simulink subsystem "Subsys_Conv_Electrical_Part_imperix_SPS"  (R2022b)
settings: Solver=VariableStepAuto  StartTime=0.0  StopTime=10.0  RelTol=1e-3
model mask{S_n=27e3, f_n=50, V_n_phph=400, V_n_grid_phph=400, V_n_dc=800, L_filter_conv_pu=[ 0.005 0.06257 ], C_filter_pu=[ 0.08437 0.03724 ], R_snubber_pu=5e6, R_on_pu=8.437e-3, C_dc_pu=5.826, P_dc_max=30e3, K_p_DC=20, K_i_DC=50}
  mask prompts: S_n "Nominal Apparent Power [VA]"; f_n "Nominal Frequency [Hz]"; V_n_phph "Nominal Converter Voltage (rms, ph-ph) [V]"; V_n_grid_phph "Nominal Grid Voltage (rms, ph-ph) [V]"; V_n_dc "DC-link voltage [V]"; L_filter_conv_pu "Impedance of Converter-Side-Inductor [ R L ] (p.u.)"; C_filter_pu "Impedance of Filter Capacitor [ R C ] (p.u.)"; R_snubber_pu "Snubber Resistance for Ideal Switches (pu)"; R_on_pu "On-State Resistance of Ideal Switches (pu)"; C_dc_pu "Capacitance of DC-link capacitors (total) (pu)"; P_dc_max "Maximum power of DC voltage source [W]"; K_p_DC "Current controller proportional gain (pu)"; K_i_DC "Current controller integral gain (pu/s)"
libraries: spsThreePhaseVIMeasurementLib x4, spsThreePhaseSeriesRLCBranchLib x3, spsSeriesRLCBranchLib x2, spsVoltageMeasurementLib x2, spsGroundLib x2, spsBreakerLib x2, spsThreePhaseBreakerLib x2, spsCurrentMeasurementLib x1, spsControlledCurrentSourceLib x1, slpidlib x1, spsUniversalBridgeLib x1
settings Model: Creator=winkens  LastModifiedBy=winkens
settings SolverCC: AlgebraicLoopSolver=TrustRegion
settings DebuggingCC: UnconnectedInputMsg=warning  UnconnectedOutputMsg=warning  UnconnectedLineMsg=warning  SFMachineParentedDataDiag=warning
settings ModelReferenceCC: EnableRefExpFcnMdlSchedulingChecks=on
settings RTWCC: DLArmComputeVersion=19.05

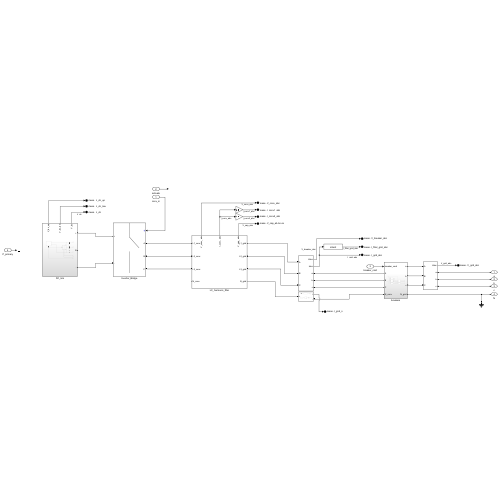
[thumbnail: Simulink's stored preview of the top-level diagram]
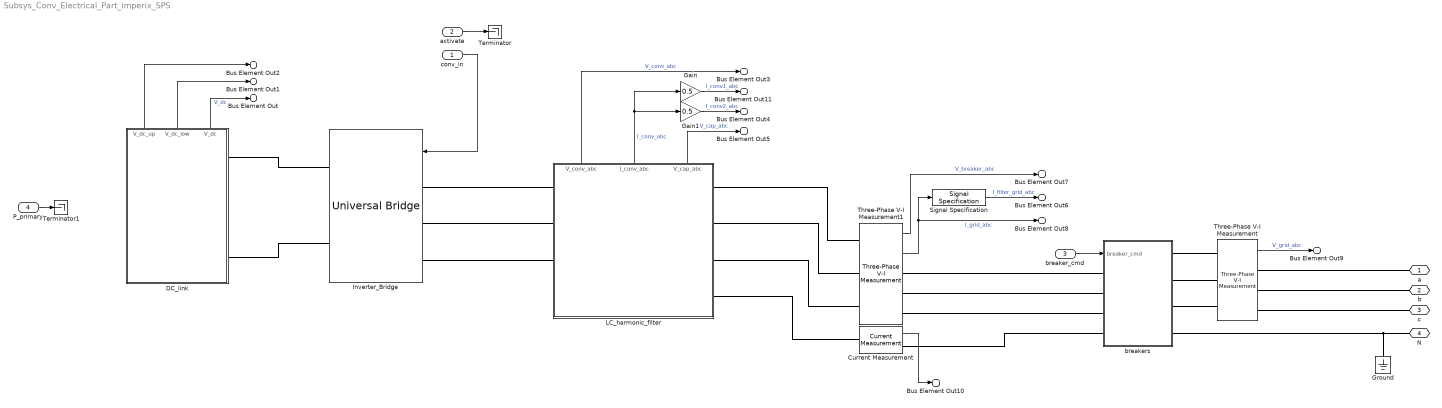
== system Subsys_Conv_Electrical_Part_imperix_SPS ==
  conv_in : Inport
  activate : Inport  Port=2
  breaker_cmd : Inport  Port=3
  P_primary : Inport  Port=4
  Current Measurement : spsCurrentMeasurementLib/Current Measurement  PhasorSimulation=off  OutputType=Complex  PSBequivalent=0
  DC_link : Subsystem  VariantControl=(default)
      settings: PortSchema="{\"entries\":[{\"content\":{\"sides\":[{\"content\":{\"connectorIds\":[]},\"type\":\"ConnectorPlacement.EquallySpacedRectSide\",\"uuid\":\"14f4955d-76e2-48f7-8123-585826302dd3\"},{\"content\":{\"connectorIds\":[\"RConn1\",\"RConn2\",\"RConn3\"],\"side\":\"RIGHT\"},\"type\":\"ConnectorPlacement.EquallySpacedRectSide\",\"uuid\":\"28c9ddee-fc07-46e8-b9fa-376576ca9eeb\"},{\"content\":{\"connectorIds\":[\"Out1\",\"Out2\",\"Out3\"],\"side\":\"TOP\"},\"type\":\"ConnectorPlacement.EquallySpacedRectSide\",\"uuid\":\"aa37790b-34b3-4fc7-a446-818c7dbc2b0a\"},{\"content\":{\"connectorIds\":[],\"side\":\"HIDDEN\"},\"type\":\"ConnectorPlacement.EquallySpacedRectSide\",\"uuid\":\"98235a86-067a-4efe-b161-de7bc0b16115\"}]},\"type\":\"ConnectorPlacement.EquallySpacedConnector\",\"uuid\":\"03b86b37-ee57-4f73-9f3c-01f441a0fa47\"}],\"packageUris\":[\"http://schema.mathworks.com/mf0/Connector/R2020b\"],\"version\":\"1.0\"}"
  Gain : Gain  Gain=0.5
  Gain1 : Gain  Gain=0.5
  Ground : spsGroundLib/Ground  LConnTagsString=a
  Inverter_Bridge : spsUniversalBridgeLib/Universal Bridge  Arms=3  SnubberResistance=R_snubber_pu*V_n_phph*V_n_phph/S_n  SnubberCapacitance=inf  Device=Ideal Switches  Ron=R_on_pu*V_n_phph*V_n_phph/S_n  Lon=0  ForwardVoltages="[  0  0  ]"  ForwardVoltage=0  GTOparameters=[ 10e-6 , 20e-6 ]  IGBTparameters=[ 1e-6 , 2e-6 ]  Measurements=None  Measurements_2=None  converterType=Rectifier
  LC_harmonic_filter : Subsystem
      settings: PortSchema="{\"entries\":[{\"content\":{\"sides\":[{\"content\":{\"connectorIds\":[\"LConn1\",\"LConn2\",\"LConn3\",\"LConn4\"]},\"type\":\"ConnectorPlacement.EquallySpacedRectSide\",\"uuid\":\"80edb88e-7f34-4d55-b68e-78bf26c6ccee\"},{\"content\":{\"connectorIds\":[\"RConn1\",\"RConn2\",\"RConn3\",\"RConn4\"],\"side\":\"RIGHT\"},\"type\":\"ConnectorPlacement.EquallySpacedRectSide\",\"uuid\":\"4bc9f7f6-7a52-4676-a444-e90f3617f1ed\"},{\"content\":{\"connectorIds\":[\"Out1\",\"Out2\",\"Out3\"],\"side\":\"TOP\"},\"type\":\"ConnectorPlacement.EquallySpacedRectSide\",\"uuid\":\"b4b56f07-3fcd-4b33-a68a-5af0641c9948\"},{\"content\":{\"connectorIds\":[],\"side\":\"HIDDEN\"},\"type\":\"ConnectorPlacement.EquallySpacedRectSide\",\"uuid\":\"916e6694-bfd6-4ec0-aa17-f6867d02ef86\"}]},\"type\":\"ConnectorPlacement.EquallySpacedConnector\",\"uuid\":\"94bee9f6-0fe3-4fcb-8152-95dcfa33148b\"}],\"packageUris\":[\"http://schema.mathworks.com/mf0/Connector/R2020b\"],\"version\":\"1.0\"}"
  Signal Specification : SignalSpecification
  Terminator : Terminator
  Terminator1 : Terminator
  Three-Phase V-I Measurement : spsThreePhaseVIMeasurementLib/Three-Phase V-I Measurement  VoltageMeasurement=phase-to-ground  SetLabelV=off  LabelV=Vabc  Vpu=off  VpuLL=off  CurrentMeasurement=no  SetLabelI=off  LabelI=Iabc  Ipu=off  Pbase=100e6  Vbase=500e3  OutputType=Complex  PhasorSimulation=off  PSBequivalent=0
  Three-Phase V-I Measurement1 : spsThreePhaseVIMeasurementLib/Three-Phase V-I Measurement  VoltageMeasurement=phase-to-ground  SetLabelV=off  LabelV=Vabc  Vpu=off  VpuLL=off  CurrentMeasurement=yes  SetLabelI=off  LabelI=Iabc  Ipu=off  Pbase=100e6  Vbase=500e3  OutputType=Complex  PhasorSimulation=off  PSBequivalent=0
  breakers : Subsystem
  a : PMIOPort  Side=Right
  b : PMIOPort  Port=2  Side=Right
  c : PMIOPort  Port=3  Side=Right
  N : PMIOPort  Port=4  Side=Right
  Bus Element Out : Outport  PortName=meas  Element=V_dc
  Bus Element Out1 : Outport  PortName=meas  Element=V_dc_low
  Bus Element Out2 : Outport  PortName=meas  Element=V_dc_up
  Bus Element Out3 : Outport  PortName=meas  Element=V_conv_abc
  Bus Element Out4 : Outport  PortName=meas  Element=I_conv2_abc
  Bus Element Out5 : Outport  PortName=meas  Element=V_cap_ab-bc-ca
  Bus Element Out6 : Outport  PortName=meas  Element=I_filter_grid_abc
  Bus Element Out7 : Outport  PortName=meas  Element=V_breaker_abc
  Bus Element Out8 : Outport  PortName=meas  Element=I_grid_abc
  Bus Element Out10 : Outport  PortName=meas  Element=I_grid_n
  Bus Element Out9 : Outport  PortName=meas  Element=V_grid_abc
  Bus Element Out11 : Outport  PortName=meas  Element=I_conv1_abc
  wires:
  Three-Phase V-I Measurement1/2 -> Signal Specification/1, Bus Element Out8/1  "I_grid_abc"
  Three-Phase V-I Measurement1/1 -> Bus Element Out7/1  "V_breaker_abc"
  LC_harmonic_filter/2(I_conv_abc) -> Gain/1, Gain1/1  "I_conv_abc"
  LC_harmonic_filter/3(V_cap_abc) -> Bus Element Out5/1  "V_cap_abc"
  DC_link/3(V_dc) -> Bus Element Out/1  "V_dc"
  Three-Phase V-I Measurement/1 -> Bus Element Out9/1  "V_grid_abc"
  LC_harmonic_filter/1(V_conv_abc) -> Bus Element Out3/1  "V_conv_abc"
  P_primary/1 -> Terminator1/1
  activate/1 -> Terminator/1
  conv_in/1 -> Inverter_Bridge/1
  Signal Specification/1 -> Bus Element Out6/1  "I_filter_grid_abc"
  DC_link/2(V_dc_low) -> Bus Element Out1/1
  DC_link/1(V_dc_up) -> Bus Element Out2/1
  breaker_cmd/1 -> breakers/1(breaker_cmd)
  Current Measurement/1 -> Bus Element Out10/1
  Gain1/1 -> Bus Element Out4/1  "I_conv2_abc"
  Gain/1 -> Bus Element Out11/1  "I_conv1_abc"
  connections:
  Ground/LConn1 -- breakers/RConn4 -- N/RConn1
  DC_link/RConn1 -- Inverter_Bridge/RConn1
  DC_link/RConn3 -- Inverter_Bridge/RConn2
  Three-Phase V-I Measurement/RConn2 -- b/RConn1
  Three-Phase V-I Measurement/RConn1 -- a/RConn1
  LC_harmonic_filter/LConn3 -- Inverter_Bridge/LConn3
  Three-Phase V-I Measurement/RConn3 -- c/RConn1
  LC_harmonic_filter/LConn1 -- Inverter_Bridge/LConn1
  LC_harmonic_filter/LConn2 -- Inverter_Bridge/LConn2
  Three-Phase V-I Measurement1/LConn1 -- LC_harmonic_filter/RConn1
  Three-Phase V-I Measurement1/LConn2 -- LC_harmonic_filter/RConn2
  Three-Phase V-I Measurement1/LConn3 -- LC_harmonic_filter/RConn3
  Three-Phase V-I Measurement/LConn1 -- breakers/RConn1
  Three-Phase V-I Measurement1/RConn1 -- breakers/LConn1
  Three-Phase V-I Measurement/LConn2 -- breakers/RConn2
  Three-Phase V-I Measurement1/RConn2 -- breakers/LConn2
  Current Measurement/LConn1 -- LC_harmonic_filter/RConn4
  Three-Phase V-I Measurement/LConn3 -- breakers/RConn3
  Three-Phase V-I Measurement1/RConn3 -- breakers/LConn3
  Current Measurement/RConn1 -- breakers/LConn4

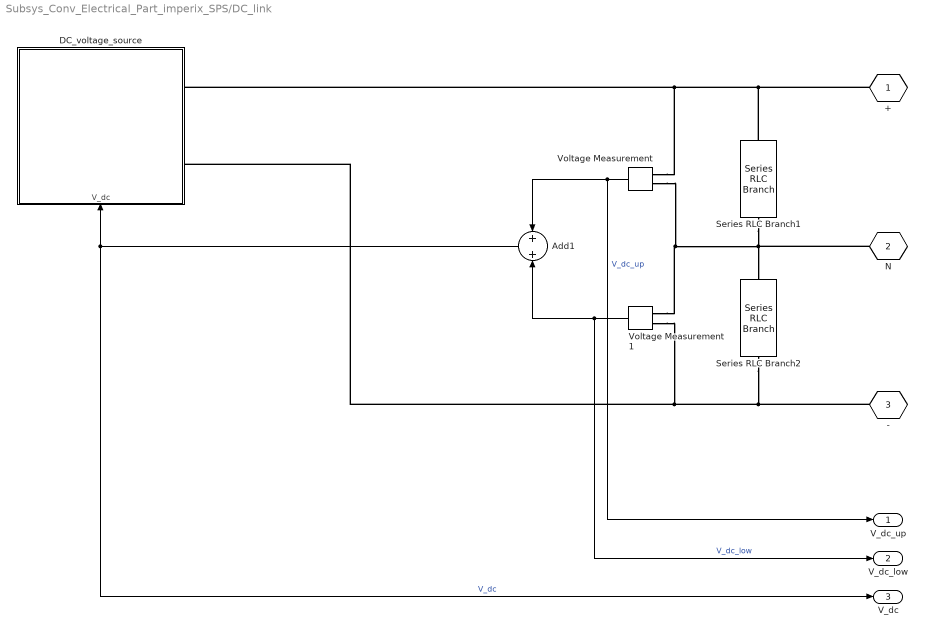
== system Subsys_Conv_Electrical_Part_imperix_SPS/DC_link ==
  Add1 : Sum  Inputs=+|+
  DC_voltage_source : Subsystem
      settings: PortSchema="{\"entries\":[{\"content\":{\"sides\":[{\"content\":{\"connectorIds\":[]},\"type\":\"ConnectorPlacement.EquallySpacedRectSide\",\"uuid\":\"a61cbdc0-cd1f-4d97-8c38-69a1c66b7135\"},{\"content\":{\"connectorIds\":[\"RConn1\",\"RConn2\"],\"side\":\"RIGHT\"},\"type\":\"ConnectorPlacement.EquallySpacedRectSide\",\"uuid\":\"763bad63-06eb-40cb-9b7c-68a57cfbd908\"},{\"content\":{\"connectorIds\":[],\"side\":\"TOP\"},\"type\":\"ConnectorPlacement.EquallySpacedRectSide\",\"uuid\":\"0a61cfd4-8f0a-43bb-bfe4-f1bce7526c22\"},{\"content\":{\"connectorIds\":[\"In1\"],\"side\":\"BOTTOM\"},\"type\":\"ConnectorPlacement.EquallySpacedRectSide\",\"uuid\":\"8fa3c57f-1077-4c84-877b-6ab8e99a2e0f\"},{\"content\":{\"connectorIds\":[],\"side\":\"HIDDEN\"},\"type\":\"ConnectorPlacement.EquallySpacedRectSide\",\"uuid\":\"ed7d5b32-63bb-486f-8710-8f53ee798462\"}]},\"type\":\"ConnectorPlacement.EquallySpacedConnector\",\"uuid\":\"0213af1d-3c14-41a0-aa43-0a8d2de349d1\"}],\"packageUris\":[\"http://schema.mathworks.com/mf0/Connector/R2020b\"],\"version\":\"1.0\"}"
  Series RLC Branch1 : spsSeriesRLCBranchLib/Series RLC Branch  LConnTagsString=__new0  RConnTagsString=__new0  BranchType=C  Resistance=1  Inductance=1e-3  SetiL0=off  InitialCurrent=0  Capacitance=2*C_dc_pu*S_n/(2*pi*f_n*V_n_phph*V_n_phph)  Setx0=on  InitialVoltage=V_n_dc/2  Measurements=None
  Series RLC Branch2 : spsSeriesRLCBranchLib/Series RLC Branch  LConnTagsString=__new0  RConnTagsString=__new0  BranchType=C  Resistance=1  Inductance=1e-3  SetiL0=off  InitialCurrent=0  Capacitance=2*C_dc_pu*S_n/(2*pi*f_n*V_n_phph*V_n_phph)  Setx0=on  InitialVoltage=V_n_dc/2  Measurements=None
  Voltage Measurement : spsVoltageMeasurementLib/Voltage Measurement  PhasorSimulation=off  OutputType=Complex  PSBequivalent=0
  Voltage Measurement1 : spsVoltageMeasurementLib/Voltage Measurement  PhasorSimulation=off  OutputType=Complex  PSBequivalent=0
  + : PMIOPort  Tag=PMCPort  Side=Right
  N : PMIOPort  Tag=PMCPort  Port=2  Side=Right
  - : PMIOPort  Tag=PMCPort  Port=3  Side=Right
  V_dc_up : Outport
  V_dc_low : Outport  Port=2
  V_dc : Outport  Port=3
  wires:
  Voltage Measurement/1 -> V_dc_up/1, Add1/1  "V_dc_up"
  Voltage Measurement1/1 -> V_dc_low/1, Add1/2  "V_dc_low"
  Add1/1 -> V_dc/1, DC_voltage_source/1(V_dc)  "V_dc"
  connections:
  Series RLC Branch2/RConn1 -- -/RConn1 -- DC_voltage_source/RConn2 -- Voltage Measurement1/LConn2
  Series RLC Branch1/RConn1 -- Voltage Measurement/LConn2 -- Voltage Measurement1/LConn1 -- Series RLC Branch2/LConn1 -- N/RConn1
  +/RConn1 -- Series RLC Branch1/LConn1 -- DC_voltage_source/RConn1 -- Voltage Measurement/LConn1

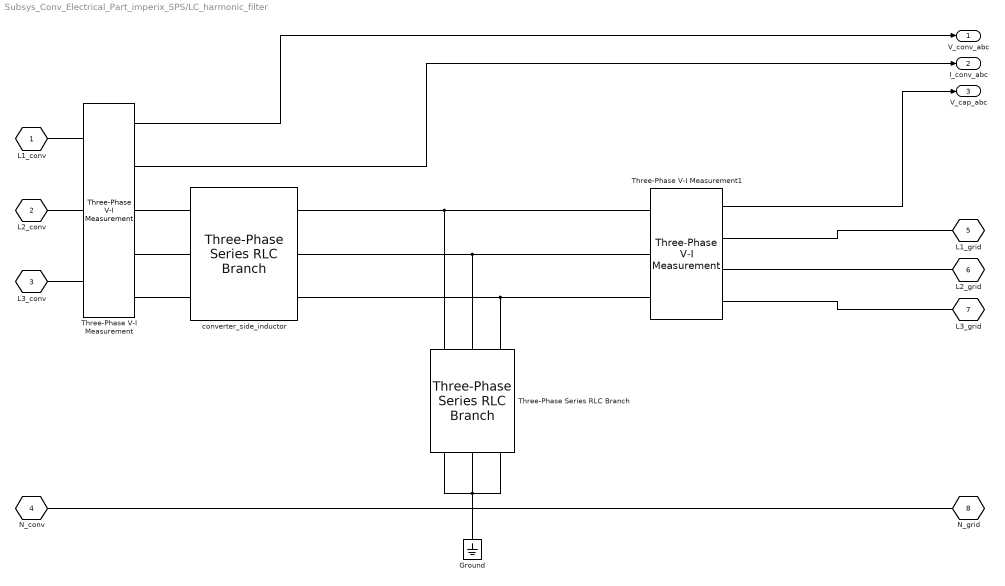
== system Subsys_Conv_Electrical_Part_imperix_SPS/LC_harmonic_filter ==
  Ground : spsGroundLib/Ground  LConnTagsString=a
  Three-Phase Series RLC Branch : spsThreePhaseSeriesRLCBranchLib/Three-Phase Series RLC Branch  LConnTagsString=A|B|C  RConnTagsString=A|B|C  BranchType=RC  Resistance=C_filter_pu(1)*V_n_phph*V_n_phph/S_n  Inductance=1e-3  Capacitance=C_filter_pu(2)*S_n/(2*pi*50*V_n_phph*V_n_phph)  Measurements=None
  Three-Phase V-I Measurement : spsThreePhaseVIMeasurementLib/Three-Phase V-I Measurement  VoltageMeasurement=phase-to-ground  SetLabelV=off  LabelV=Vabc  Vpu=off  VpuLL=off  CurrentMeasurement=yes  SetLabelI=off  LabelI=Iabc  Ipu=off  Pbase=100e6  Vbase=500e3  OutputType=Complex  PhasorSimulation=off  PSBequivalent=0
  Three-Phase V-I Measurement1 : spsThreePhaseVIMeasurementLib/Three-Phase V-I Measurement  VoltageMeasurement=phase-to-phase  SetLabelV=off  LabelV=Vabc  Vpu=off  VpuLL=off  CurrentMeasurement=no  SetLabelI=off  LabelI=Iabc  Ipu=off  Pbase=100e6  Vbase=500e3  OutputType=Complex  PhasorSimulation=off  PSBequivalent=0
  converter_side_inductor : spsThreePhaseSeriesRLCBranchLib/Three-Phase Series RLC Branch  LConnTagsString=A|B|C  RConnTagsString=A|B|C  BranchType=RL  Resistance=L_filter_conv_pu(1)*V_n_phph*V_n_phph/S_n  Inductance=L_filter_conv_pu(2)*V_n_phph*V_n_phph/(2*pi*f_n*S_n)  Capacitance=1e-6  Measurements=None
  L1_conv : PMIOPort  Tag=PMCPort  Side=Left
  L2_conv : PMIOPort  Tag=PMCPort  Port=2  Side=Left
  L3_conv : PMIOPort  Tag=PMCPort  Port=3  Side=Left
  N_conv : PMIOPort  Tag=PMCPort  Port=4  Side=Left
  L1_grid : PMIOPort  Tag=PMCPort  Port=5  Side=Right
  L2_grid : PMIOPort  Tag=PMCPort  Port=6  Side=Right
  L3_grid : PMIOPort  Tag=PMCPort  Port=7  Side=Right
  N_grid : PMIOPort  Tag=PMCPort  Port=8  Side=Right
  V_conv_abc : Outport
  I_conv_abc : Outport  Port=2
  V_cap_abc : Outport  Port=3
  wires:
  Three-Phase V-I Measurement/1 -> V_conv_abc/1
  Three-Phase V-I Measurement1/1 -> V_cap_abc/1
  Three-Phase V-I Measurement/2 -> I_conv_abc/1
  connections:
  converter_side_inductor/RConn2 -- Three-Phase Series RLC Branch/LConn2 -- Three-Phase V-I Measurement1/LConn2
  converter_side_inductor/RConn3 -- Three-Phase Series RLC Branch/LConn3 -- Three-Phase V-I Measurement1/LConn3
  converter_side_inductor/RConn1 -- Three-Phase V-I Measurement1/LConn1 -- Three-Phase Series RLC Branch/LConn1
  Three-Phase Series RLC Branch/RConn2 -- Ground/LConn1 -- N_grid/RConn1 -- N_conv/RConn1 -- Three-Phase Series RLC Branch/RConn1 -- Three-Phase Series RLC Branch/RConn3
  Three-Phase V-I Measurement/RConn3 -- converter_side_inductor/LConn3
  Three-Phase V-I Measurement/RConn2 -- converter_side_inductor/LConn2
  Three-Phase V-I Measurement/RConn1 -- converter_side_inductor/LConn1
  Three-Phase V-I Measurement/LConn3 -- L3_conv/RConn1
  Three-Phase V-I Measurement/LConn2 -- L2_conv/RConn1
  Three-Phase V-I Measurement/LConn1 -- L1_conv/RConn1
  Three-Phase V-I Measurement1/RConn1 -- L1_grid/RConn1
  Three-Phase V-I Measurement1/RConn2 -- L2_grid/RConn1
  Three-Phase V-I Measurement1/RConn3 -- L3_grid/RConn1

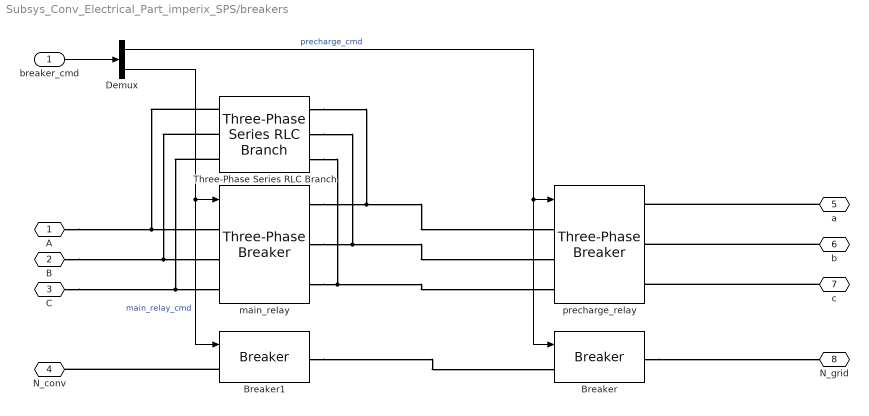
== system Subsys_Conv_Electrical_Part_imperix_SPS/breakers ==
  breaker_cmd : Inport
  Breaker : spsBreakerLib/Breaker  InitialState=0  SwitchingTimes="[1/60  5/60]"  External=on  BreakerResistance=0.001  SnubberResistance=1e6  SnubberCapacitance=inf  Measurements=None  MoreParameters=on  NoBreakLoop=off
  Breaker1 : spsBreakerLib/Breaker  InitialState=0  SwitchingTimes="[1/60  5/60]"  External=on  BreakerResistance=0.001  SnubberResistance=1e6  SnubberCapacitance=inf  Measurements=None  MoreParameters=on  NoBreakLoop=off
  Demux : Demux  Outputs=2
  Three-Phase Series RLC Branch : spsThreePhaseSeriesRLCBranchLib/Three-Phase Series RLC Branch  LConnTagsString=A|B|C  RConnTagsString=A|B|C  BranchType=R  Resistance=47  Inductance=1e-3  Capacitance=1e-6  Measurements=None
  main_relay : spsThreePhaseBreakerLib/Three-Phase Breaker  InitialState=open  SwitchA=on  SwitchB=on  SwitchC=on  SwitchTimes="[1/60  5/60]"  External=on  BreakerResistance=0.001  SnubberResistance=1e6  SnubberCapacitance=inf  Measurements=None
  precharge_relay : spsThreePhaseBreakerLib/Three-Phase Breaker  InitialState=open  SwitchA=on  SwitchB=on  SwitchC=on  SwitchTimes="[1/60  5/60]"  External=on  BreakerResistance=0.001  SnubberResistance=1e6  SnubberCapacitance=inf  Measurements=None
  A : PMIOPort  Side=Left
  B : PMIOPort  Port=2  Side=Left
  C : PMIOPort  Port=3  Side=Left
  N_conv : PMIOPort  Port=4  Side=Left
  a : PMIOPort  Port=5  Side=Right
  b : PMIOPort  Port=6  Side=Right
  c : PMIOPort  Port=7  Side=Right
  N_grid : PMIOPort  Port=8  Side=Right
  wires:
  Demux/1 -> Breaker/1, precharge_relay/1  "precharge_cmd"
  breaker_cmd/1 -> Demux/1
  Demux/2 -> Breaker1/1, main_relay/1  "main_relay_cmd"
  connections:
  Breaker1/LConn1 -- N_conv/RConn1
  b/RConn1 -- precharge_relay/RConn2
  B/RConn1 -- Three-Phase Series RLC Branch/LConn2 -- main_relay/LConn2
  A/RConn1 -- main_relay/LConn1 -- Three-Phase Series RLC Branch/LConn1
  a/RConn1 -- precharge_relay/RConn1
  c/RConn1 -- precharge_relay/RConn3
  C/RConn1 -- Three-Phase Series RLC Branch/LConn3 -- main_relay/LConn3
  Breaker/RConn1 -- N_grid/RConn1
  main_relay/RConn1 -- Three-Phase Series RLC Branch/RConn1 -- precharge_relay/LConn1
  main_relay/RConn2 -- Three-Phase Series RLC Branch/RConn2 -- precharge_relay/LConn2
  main_relay/RConn3 -- Three-Phase Series RLC Branch/RConn3 -- precharge_relay/LConn3
  Breaker1/RConn1 -- Breaker/LConn1

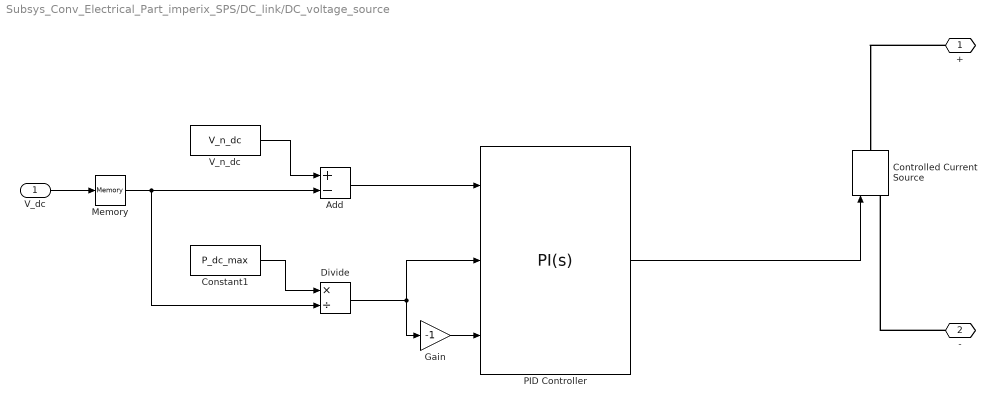
== system Subsys_Conv_Electrical_Part_imperix_SPS/DC_link/DC_voltage_source ==
  V_dc : Inport
  Add : Sum  Inputs=+-
  Constant1 : Constant  Value=P_dc_max
  Controlled Current Source : spsControlledCurrentSourceLib/Controlled Current Source  Initialize=on  Source_Type=DC  Amplitude=0  Phase=0  Frequency=0  Measurements=None
  Divide : Product  Inputs=*/
  Gain : Gain  Gain=-1
  Memory : Memory  InitialCondition=V_n_dc
  PID Controller : slpidlib/PID Controller  Controller=PI  Form=Parallel  TimeDomain=Continuous-time  UseExternalTs=off  SampleTime=-1  IntegratorMethod=Forward Euler  FilterMethod=Forward Euler  ControllerParametersSource=internal  P=K_p_DC*S_n/(V_n_phph*V_n_phph)  I=K_i_DC*S_n/(V_n_phph*V_n_phph)  UseKiTs=off  D=0  N=100  UseFilter=on  TunerSelectOption=Transfer Function Based (PID Tuner App)  InitialConditionSource=internal  InitialConditionForIntegrator=0  InitialConditionForFilter=0  DifferentiatorICPrevScaledInput=0  ExternalReset=none  TrackingMode=off  Kt=1  LimitOutput=on  SatLimitsSource=external  UpperSaturationLimit=inf  LowerSaturationLimit=-inf  LinearizeAsGain=on  AntiWindupMode=clamping  Kb=1  LimitIntegrator=off  UpperIntegratorSaturationLimit=inf  LowerIntegratorSaturationLimit=-inf  POutMin=[]  POutMax=[]  IOutMin=[]  IOutMax=[]  DOutMin=[]  DOutMax=[]  NOutMin=[]  NOutMax=[]  SumOutMin=[]  SumOutMax=[]  SaturationOutMin=[]  SaturationOutMax=[]  PParamMin=[]  PParamMax=[]  IParamMin=[]  IParamMax=[]  DParamMin=[]  DParamMax=[]  NParamMin=[]  NParamMax=[]  KbParamMin=[]  KbParamMax=[]  KtParamMin=[]  KtParamMax=[]  KbOutMin=[]  KbOutMax=[]  KtOutMin=[]  KtOutMax=[]  IntegratorOutMin=[]  IntegratorOutMax=[]  FilterOutMin=[]  FilterOutMax=[]  SumI1OutMin=[]  SumI1OutMax=[]  SumI2OutMin=[]  SumI2OutMax=[]  SumI3OutMin=[]  SumI3OutMax=[]  SumI4OutMin=[]  SumI4OutMax=[]  SumDOutMin=[]  SumDOutMax=[]  DifferentiatorOutMin=[]  DifferentiatorOutMax=[]  FilterDiffOutCoefMin=[]  FilterDiffOutCoefMax=[]  ReciprocalOutMin=[]  ReciprocalOutMax=[]  SumDenOutMin=[]  SumDenOutMax=[]  SumNumOutMin=[]  SumNumOutMax=[]  DivideOutMin=[]  DivideOutMax=[]  UdiffTsProdOutMin=[]  UdiffTsProdOutMax=[]  NTsProdOutMin=[]  NTsProdOutMax=[]  UintegralTsProdOutMin=[]  UintegralTsProdOutMax=[]  UngainTsProdOutMin=[]  UngainTsProdOutMax=[]  ClampingZeroOutDataTypeStr=Inherit: Inherit via back propagation  ClampingZeroOutMin=[]  ClampingZeroOutMax=[]  FilterDenConstantOutDataTypeStr=Inherit: Inherit via back propagation  FilterDenConstantOutMin=[]  FilterDenConstantOutMax=[]  PCopyOutDataTypeStr=Inherit: Inherit via back propagation  PCopyOutMin=[]  PCopyOutMax=[]  NCopyOutDataTypeStr=Inherit: Inherit via back propagation  NCopyOutMin=[]  NCopyOutMax=[]  IntegratorContinuousStateAttributes=''  IntegratorStateMustResolveToSignalObject=off  IntegratorRTWStateStorageClass=Auto  FilterContinuousStateAttributes=''  FilterStateMustResolveToSignalObject=off  FilterRTWStateStorageClass=Auto  ParallelPVariant=InternalParameters  IdealPVariant=Disabled  IVariant=InternalParameters  DVariant=Disabled  IntegratorVariant=Continuous  SatVariant=External  AWVariant=ContClampingParallel  PCopyVariant=Disabled  TRVariant=Disabled  FdbkBlocksVariant=Forward  IdealPFdbkVariant=Disabled  SatFdbkVariant=Disabled  DerivativeFilterVariant=Disabled  NVariant=Disabled  NCopyVariant=Disabled_SignalSpec  FilterICVariant=Disabled  IntegratorICVariant=InternalICs  ExternalResetVariant=Disabled  TRSumVariant=Passthrough  SumFdbkVariant=Disabled  SumVariant=Sum_PI  TsampFilterVariant=InternalTs  TsampNgainVariant=Passthrough  TsampIntegralVariant=Passthrough  ExternalSaturationOutDataTypeStr=Inherit: Same as second input
  V_n_dc : Constant  Value=V_n_dc
  + : PMIOPort  Side=Right
  - : PMIOPort  Port=2  Side=Right
  wires:
  Divide/1 -> Gain/1, PID Controller/2
  V_n_dc/1 -> Add/1
  Add/1 -> PID Controller/1
  Gain/1 -> PID Controller/3
  PID Controller/1 -> Controlled Current Source/1
  V_dc/1 -> Memory/1
  Constant1/1 -> Divide/1
  Memory/1 -> Add/2, Divide/2
  connections:
  +/RConn1 -- Controlled Current Source/RConn1
  -/RConn1 -- Controlled Current Source/LConn1
